simulink model "source_binaire"  (R2023b)
settings: Solver=VariableStepAuto  StartTime=0.0  StopTime=20  RelTol=1e-3
values from neighbouring files (symbols this model uses):
  P = parametres_perso('LABBE Emmy')    [P2_Q11_LZ78_convergence.m]    (also in P2_Q1_source_binaire_simulation.m; P2_Q7_extension_source.m; P3_Q10_parametres_integration.m; P3_Q11_variance_integrateur.m)
  Tb = 1;')    [LANCER_TP_COMPLET.m]    (also in P2_Q1_source_binaire_simulation.m = 1; P3_Q10_parametres_integration.m = 1; P3_Q11_variance_integrateur.m = 1; P3_Q12_TEB.m = 1)
libraries: simulink x1
settings Model: Creator=e2202522  LastModifiedBy=e2202522

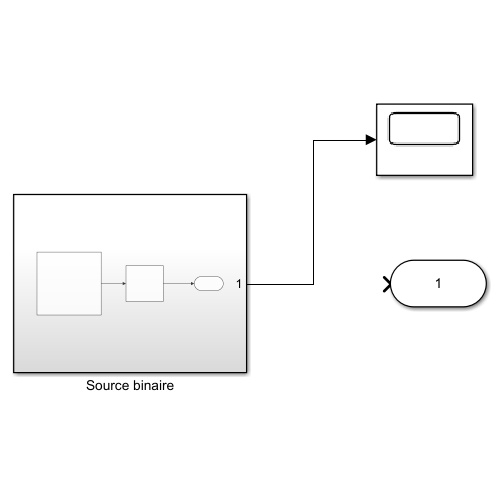
[thumbnail: Simulink's stored preview of the top-level diagram]
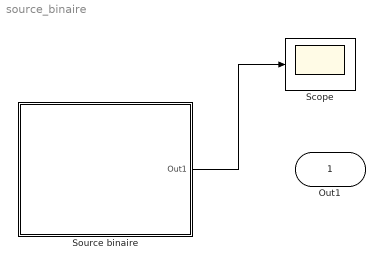
== system source_binaire ==
  Scope : Scope
  Source binaire : Subsystem
  Out1 : Outport
  wires:
  Source binaire/1(Out1) -> Scope/1

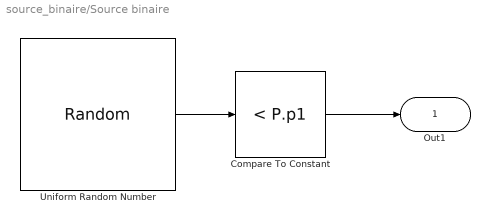
== system source_binaire/Source binaire ==
  Compare To Constant : simulink/Logic and Bit Operations/Compare To Constant  relop=<  const=P.p1  OutDataTypeStr=boolean
  Uniform Random Number : UniformRandomNumber  Minimum=0  Seed=P.graine  SampleTime=Tb
  Out1 : Outport
  wires:
  Compare To Constant/1 -> Out1/1
  Uniform Random Number/1 -> Compare To Constant/1
